simulink model "F16Trim6DOF"  (R2025b)
settings: Solver=ode4  StartTime=0  StopTime=P6dof.tFinal  FixedStep=P6dof.dt  RelTol=1e-3
InitFcn:
  | if ~exist('P6dof', 'var'), P6dof = vital.slx.trim6dofSetup(); end
  | vital.slx.f16LoadsCg('setup', P6dof);
StopFcn:
  | if exist('sim6dof', 'var') && exist('P6dof', 'var') && P6dof.plot
  |     vital.slx.plotTrim6dof(sim6dof, P6dof);
  | end
undefined symbols (not defined in the file): P6dof
libraries: aerolibasang x3, aerolibatmos2 x1
settings Model: Creator=krish  LastModifiedBy=krish
settings DataIOCC: SaveFormat=StructureWithTime  SignalLogging=off  ReturnWorkspaceOutputs=off
settings DebuggingCC: AlgebraicLoopMsg=error

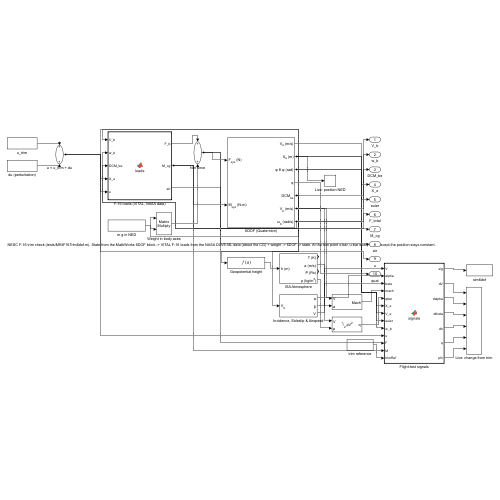
[thumbnail: Simulink's stored preview of the top-level diagram]
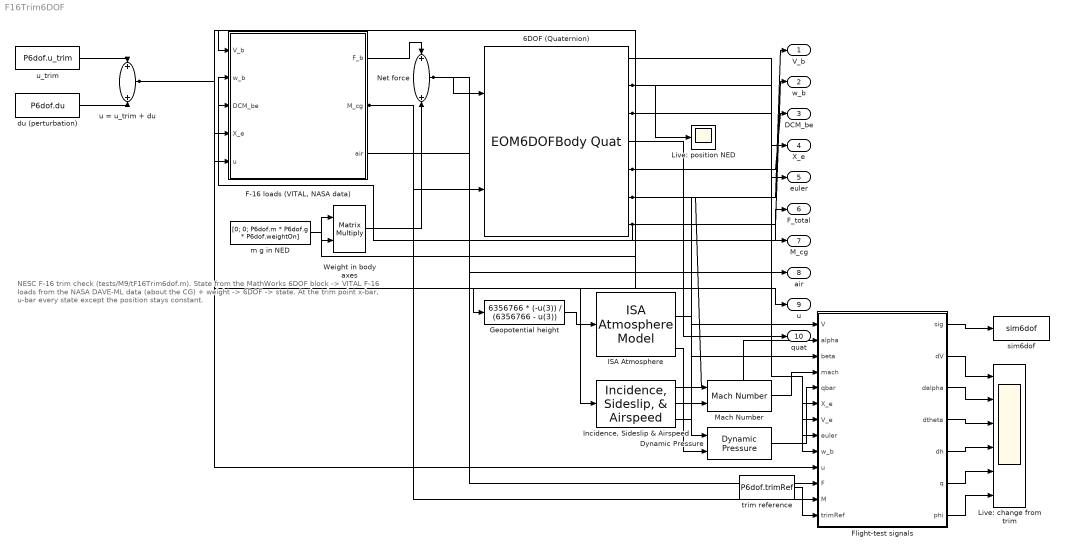
== system F16Trim6DOF ==
  note: NESC F-16 trim check (tests/M9/tF16Trim6dof.m). State from the MathWorks 6DOF block -> VITAL F-16 loads from the NASA DAVE-ML data (about the CG) + weight -> 6DOF -> state. At the trim point x-bar, u-bar every state except the position stays constant.
  6DOF (Quaternion) : EOM6DOFBodyQuat  xme_0=P6dof.Xe0'  Vm_0=P6dof.Vb0'  eul_0=P6dof.eul0'  pm_0=P6dof.w0'  mass_0=P6dof.m  inertia=P6dof.J
  Dynamic Pressure : aerolibasang/Dynamic Pressure
  "F-16 loads (VITAL, NASA data)" : MATLAB Function  TreatAsAtomicUnit=on
  Flight-test signals : MATLAB Function  TreatAsAtomicUnit=on
  Geopotential height : Fcn  Expr=6356766 * (-u(3)) / (6356766 - u(3))
  ISA Atmosphere : aerolibatmos2/ISA Atmosphere Model  useExtended=off  action=None  custom=off  viscosityOut=off  g=9.80665  gamma=1.4  R=287.0531  L=0.0065  h_trop=11000  h_strat=20000  rho0=1.225  P0=101325  T0=288.15  h0=0  S=110.4  Tref=273.15  muref=1.716e-5
  "Incidence, Sideslip & Airspeed" : aerolibasang/Incidence, Sideslip, & Airspeed
  Live: change from trim : Scope  NumInputPorts=6
      settings: Title=change from trim: dV (ft/s)  ActiveDisplayYMinimum=-1  ActiveDisplayYMaximum=1
  Live: position NED : Scope
  Mach Number : aerolibasang/Mach Number
  Net force : Sum
  Weight in body axes : Product  Inputs=**  Multiplication=Matrix(*)
  du (perturbation) : FromWorkspace  VariableName=P6dof.du  SampleTime=P6dof.dt  Interpolate=off  OutputAfterFinalValue=Holding final value
  m g in NED : Constant  Value=[0; 0; P6dof.m * P6dof.g * P6dof.weightOn]
  sim6dof : ToWorkspace  VariableName=sim6dof  SaveFormat=Structure With Time  SampleTime=-1
  trim reference : Constant  Value=P6dof.trimRef
  u = u_trim + du : Sum
  u_trim : Constant  Value=P6dof.u_trim
  V_b : Outport
  w_b : Outport  Port=2
  DCM_be : Outport  Port=3
  X_e : Outport  Port=4
  euler : Outport  Port=5
  F_total : Outport  Port=6
  M_cg : Outport  Port=7
  air : Outport  Port=8
  u : Outport  Port=9
  quat : Outport  Port=10
  wires:
  u_trim/1 -> u = u_trim + du/1
  du (perturbation)/1 -> u = u_trim + du/2
  6DOF (Quaternion)/6 -> "F-16 loads (VITAL, NASA data)"/1(V_b), V_b/1, "Incidence, Sideslip & Airspeed"/1, Mach Number/1, Dynamic Pressure/1
  6DOF (Quaternion)/7 -> "F-16 loads (VITAL, NASA data)"/2(w_b), w_b/1, Flight-test signals/9(w_b)
  6DOF (Quaternion)/5 -> "F-16 loads (VITAL, NASA data)"/3(DCM_be), Weight in body axes/1, DCM_be/1
  6DOF (Quaternion)/2 -> "F-16 loads (VITAL, NASA data)"/4(X_e), X_e/1, Live: position NED/1, Geopotential height/1, Flight-test signals/6(X_e)
  u = u_trim + du/1 -> "F-16 loads (VITAL, NASA data)"/5(u), u/1, Flight-test signals/10(u)
  m g in NED/1 -> Weight in body axes/2
  "F-16 loads (VITAL, NASA data)"/1(F_b) -> Net force/1
  Weight in body axes/1 -> Net force/2
  Net force/1 -> 6DOF (Quaternion)/1, F_total/1, Flight-test signals/11(F)
  "F-16 loads (VITAL, NASA data)"/2(M_cg) -> 6DOF (Quaternion)/2, M_cg/1, Flight-test signals/12(M)
  6DOF (Quaternion)/3 -> euler/1, Flight-test signals/8(euler)
  "F-16 loads (VITAL, NASA data)"/3(air) -> air/1
  6DOF (Quaternion)/4 -> quat/1
  Geopotential height/1 -> ISA Atmosphere/1
  ISA Atmosphere/2 -> Mach Number/2
  ISA Atmosphere/4 -> Dynamic Pressure/2
  "Incidence, Sideslip & Airspeed"/3 -> Flight-test signals/1(V)
  "Incidence, Sideslip & Airspeed"/1 -> Flight-test signals/2(alpha)
  "Incidence, Sideslip & Airspeed"/2 -> Flight-test signals/3(beta)
  Mach Number/1 -> Flight-test signals/4(mach)
  Dynamic Pressure/1 -> Flight-test signals/5(qbar)
  6DOF (Quaternion)/1 -> Flight-test signals/7(V_e)
  trim reference/1 -> Flight-test signals/13(trimRef)
  Flight-test signals/1(sig) -> sim6dof/1
  Flight-test signals/2(dV) -> Live: change from trim/1
  Flight-test signals/3(dalpha) -> Live: change from trim/2
  Flight-test signals/4(dtheta) -> Live: change from trim/3
  Flight-test signals/5(dh) -> Live: change from trim/4
  Flight-test signals/6(q) -> Live: change from trim/5
  Flight-test signals/7(phi) -> Live: change from trim/6

== matlab function F16Trim6DOF/Flight-test signals ==
  data: V input; alpha input; beta input; mach input; qbar input; X_e input; V_e input; euler input; w_b input; u input; sig output; F input; M input; trimRef input; dV output; dalpha output; dtheta output; dh output; q output; phi output
function [sig, dV, dalpha, dtheta, dh, q, phi] = signals(V, alpha, beta, mach, qbar, X_e, V_e, euler, w_b, u, F, M, trimRef)
%SIGNALS  The flight-test signals of this run, all from Simulink blocks (SI, rad):
%   sig = [V alpha beta Mach qbar h hdot phi theta psi p q r xN xE de da dr throttle Fx Fy Fz L M N]
%   and, for the live scope, the change from the trim value trimRef = [V alpha theta h]
%   (ft/s, deg, deg, ft) plus q (deg/s) and phi (deg).
h = -X_e(3); hdot = -V_e(3);
sig = [V; alpha; beta; mach; qbar; h; hdot; euler(:); w_b(:); X_e(1); X_e(2); u(:); F(:); M(:)];
dV = (V - trimRef(1)) / 0.3048; dalpha = (alpha - trimRef(2)) * 180 / pi;
dtheta = (euler(2) - trimRef(3)) * 180 / pi; dh = (h - trimRef(4)) / 0.3048;
q = w_b(2) * 180 / pi; phi = euler(1) * 180 / pi;
end

== matlab function F16Trim6DOF/F-16 loads (VITAL, NASA data) ==
  data: V_b input; w_b input; DCM_be input; X_e input; u input; F_b output; M_cg output; air output
function [F_b, M_cg, air] = loads(V_b, w_b, DCM_be, X_e, u)
%LOADS  Aero + thrust of the NESC F-16 about the CG, body axes (no weight).
%   vital.slx.f16LoadsCg evaluates the VITAL AircraftModel built from the NASA
%   DAVE-ML data objects. air = [V alpha beta Mach qbar h].
coder.extrinsic('vital.slx.f16LoadsCg');
F_b = zeros(3, 1); M_cg = zeros(3, 1); air = zeros(6, 1);
[F_b, M_cg, air] = vital.slx.f16LoadsCg(V_b, w_b, DCM_be, X_e, u);
end
